simulink model "student_model_animation_2024a"  (R2024a)
settings: Solver=VariableStepAuto  StartTime=0.0  StopTime=t_sim  RelTol=1e-3
values from neighbouring files (symbols this model uses):
  L = 1    [student_lab3_model_ref.m]
undefined symbols (not defined in the file or in its folder): X, Y, Z
libraries: sm_lib x13, nesl_utility x3
settings Model: Creator=trome3  LastModifiedBy=trome3
settings ConfigComp: CovBoundaryAbsTol=1.0e-5

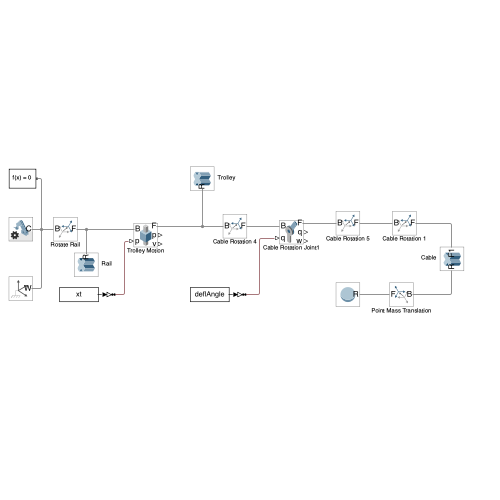
[thumbnail: Simulink's stored preview of the top-level diagram]
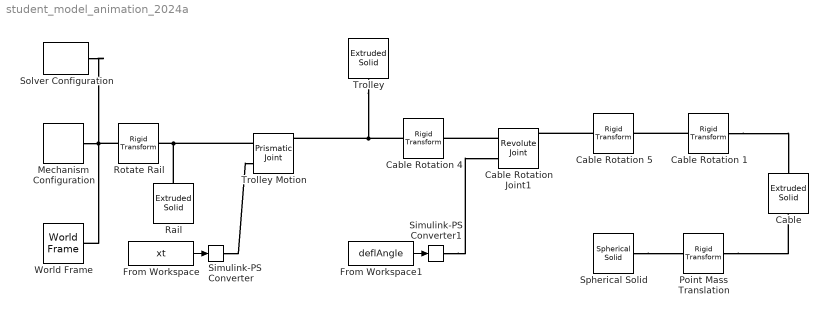
== system student_model_animation_2024a ==
  Cable : sm_lib/Body Elements/Extruded Solid  ExtrusionType=General  PolygonNumSides=1  PolygonOuterRadius=1  PolygonOuterRadiusUnits=m  ExportEntireGeometry=off  ExtrusionCrossSection=[1 1; -1 1; -1 -1; 1 -1]  ExtrusionCrossSectionUnits=cm  ExportConvexHullGeometry=off  ExtrusionLength=L  ExtrusionLengthUnits=m  InertiaType=Custom  BasedOnType=Density  Density=1000  DensityUnits=kg/m^3  Mass=0  MassUnits=kg  CenterOfMass=[0 0 0]  CenterOfMassUnits=m  MomentsOfInertia=[0 0 0]  MomentsOfInertiaUnits=kg*m^2  ProductsOfInertia=[0 0 0]  ProductsOfInertiaUnits=kg*m^2  GraphicType=FromGeometry  MarkerShape=Sphere  MarkerSize=10  GraphicVisPropType=SimpleVisualProperties  GraphicDiffuseColor=[0.5 0.5 0.5]  GraphicOpacity=1  GraphicSpecularColor=[0.5 0.5 0.5 1.0]  GraphicAmbientColor=[0.15 0.15 0.15 1.0]  GraphicEmissiveColor=[0.0 0.0 0.0 1.0]  GraphicShininess=75  DoExposeReferenceFrame=on  SerializedFrames=|
      | <Frames>
      | 
      |   <Frame>
      |     <Id>Frame1</Id>
      |     <Value>
      |       <Name>F1</Name>
      |       <Origin>
      |         <Source>GeometricFeature</Source>
      |         <FeatureName>top surface</FeatureName>
      |       </Origin>
      |       <PrimaryAxis>
      |         <DefinedDirection>+Z</DefinedDirection>
      |         <Source>ReferenceFrame</Source>
      |         <SourceDirection>+Z</SourceDirection>
      |         <FeatureName></FeatureName>
      |       </PrimaryAxis>
      |       <SecondaryAxis>
      |         <DefinedDirection>+X</DefinedDirection>
      |         <Source>ReferenceFrame</Source>
      |         <SourceDirection>+X</SourceDirection>
      |         <FeatureName></FeatureName>
      |       </SecondaryAxis>
      |     </Value>
      |   </Frame>
      | 
      | </Frames>
  Cable Rotation 1 : sm_lib/Frames and Transforms/Rigid Transform  RotationMethod=RotationSequence  FollAlignAxisA=+X  BaseAlignAxisA=+Y  FollAlignAxisB=+Y  BaseAlignAxisB=+Z  RotationStandardAxis=+Z  RotationAngle=0  RotationAngleUnits=deg  RotationArbitraryAxis=[0 0 1]  RotationSequenceAxes=FollowerAxes  RotationSequence=ZYX  RotationSequenceAngles=[0 0 -90]  RotationSequenceAnglesUnits=deg  RotationMatrix=[1 0 0;0 1 0;0 0 1]  Quaternion=[1 0 0 0]  TranslationMethod=None  TranslationCartesianOffset=[0 0 0]  TranslationCartesianOffsetUnits=m  TranslationStandardAxis=+Z  TranslationStandardOffset=L/2  TranslationStandardOffsetUnits=m  TranslationROffset=0  TranslationROffsetUnits=m  TranslationThetaOffset=0  TranslationThetaOffsetUnits=deg  TranslationZOffset=0  TranslationZOffsetUnits=m
  Cable Rotation 4 : sm_lib/Frames and Transforms/Rigid Transform  RotationMethod=RotationSequence  FollAlignAxisA=+X  BaseAlignAxisA=+Y  FollAlignAxisB=+Y  BaseAlignAxisB=+Z  RotationStandardAxis=+X  RotationAngle=0  RotationAngleUnits=deg  RotationArbitraryAxis=[0 0 1]  RotationSequenceAxes=FollowerAxes  RotationSequence=XYZ  RotationSequenceAngles=[0 90 0]  RotationSequenceAnglesUnits=deg  RotationMatrix=[1 0 0;0 1 0;0 0 1]  Quaternion=[1 0 0 0]  TranslationMethod=None  TranslationCartesianOffset=[0 0 0]  TranslationCartesianOffsetUnits=m  TranslationStandardAxis=+Z  TranslationStandardOffset=L/2  TranslationStandardOffsetUnits=m  TranslationROffset=0  TranslationROffsetUnits=m  TranslationThetaOffset=0  TranslationThetaOffsetUnits=deg  TranslationZOffset=0  TranslationZOffsetUnits=m
  Cable Rotation 5 : sm_lib/Frames and Transforms/Rigid Transform  RotationMethod=RotationSequence  FollAlignAxisA=+X  BaseAlignAxisA=+Y  FollAlignAxisB=+Y  BaseAlignAxisB=+Z  RotationStandardAxis=+X  RotationAngle=0  RotationAngleUnits=deg  RotationArbitraryAxis=[0 0 1]  RotationSequenceAxes=FollowerAxes  RotationSequence=ZYX  RotationSequenceAngles=[0 -90 0]  RotationSequenceAnglesUnits=deg  RotationMatrix=[1 0 0;0 1 0;0 0 1]  Quaternion=[1 0 0 0]  TranslationMethod=None  TranslationCartesianOffset=[0 0 0]  TranslationCartesianOffsetUnits=m  TranslationStandardAxis=+Z  TranslationStandardOffset=L/2  TranslationStandardOffsetUnits=m  TranslationROffset=0  TranslationROffsetUnits=m  TranslationThetaOffset=0  TranslationThetaOffsetUnits=deg  TranslationZOffset=0  TranslationZOffsetUnits=m
  Cable Rotation Joint1 : sm_lib/Joints/Revolute Joint  JointMode=Normal  CompositeWrenchDir=FollowerOnBase  CompositeWrenchFrame=BaseFrame  SenseConstraintForce=off  SenseConstraintTorque=off  SenseTotalForce=off  SenseTotalTorque=off  PositionTargetSpecify=off  PositionTargetPriority=High  PositionTargetValue=20  PositionTargetValueUnits=deg  VelocityTargetSpecify=off  VelocityTargetPriority=High  VelocityTargetValue=0  VelocityTargetValueUnits=deg/s  EquilibriumPosition=0  EquilibriumPositionUnits=deg  SpringStiffness=0  SpringStiffnessUnits=N*m/deg  DampingCoefficient=0  DampingCoefficientUnits=N*m/(deg/s)  LowerLimitSpecify=off  LowerLimitBound=-90  LowerLimitBoundUnits=deg  LowerLimitStiffness=1e4  LowerLimitStiffnessUnits=N*m/deg  LowerLimitDamping=10  LowerLimitDampingUnits=N*m/(deg/s)  LowerLimitTransitionRegionWidth=0.1  LowerLimitTransitionRegionWidthUnits=deg  UpperLimitSpecify=off  UpperLimitBound=90  UpperLimitBoundUnits=deg  UpperLimitStiffness=1e4  UpperLimitStiffnessUnits=N*m/deg  UpperLimitDamping=10  UpperLimitDampingUnits=N*m/(deg/s)  UpperLimitTransitionRegionWidth=0.1  UpperLimitTransitionRegionWidthUnits=deg  TorqueActuationMode=ComputedTorque  MotionActuationMode=InputMotion  SensePosition=on  SenseVelocity=on  SenseAcceleration=off  SenseTorqueForce=off  SenseLowerLimitTorqueForce=off  SenseUpperLimitTorqueForce=off
  From Workspace : FromWorkspace  VariableName=xt
  From Workspace1 : FromWorkspace  VariableName=deflAngle
  Mechanism Configuration : sm_lib/Utilities/Mechanism Configuration  UniformGravity=Constant  GravityVector=[0 0 -9.80665]  GravityVectorUnits=m/s^2  LinearizationDelta=0.001  JointModeTransitionNonlinearIterations=2
  Point Mass Translation : sm_lib/Frames and Transforms/Rigid Transform  RotationMethod=None  FollAlignAxisA=+X  BaseAlignAxisA=+Y  FollAlignAxisB=+Y  BaseAlignAxisB=+Z  RotationStandardAxis=+X  RotationAngle=0  RotationAngleUnits=deg  RotationArbitraryAxis=[0 0 1]  RotationSequenceAxes=FollowerAxes  RotationSequence=ZYX  RotationSequenceAngles=[0 -90 -90]  RotationSequenceAnglesUnits=deg  RotationMatrix=[1 0 0;0 1 0;0 0 1]  Quaternion=[1 0 0 0]  TranslationMethod=StandardAxis  TranslationCartesianOffset=[0 0 0]  TranslationCartesianOffsetUnits=m  TranslationStandardAxis=+Z  TranslationStandardOffset=-L/2  TranslationStandardOffsetUnits=m  TranslationROffset=0  TranslationROffsetUnits=m  TranslationThetaOffset=0  TranslationThetaOffsetUnits=deg  TranslationZOffset=0  TranslationZOffsetUnits=m
  Rail : sm_lib/Body Elements/Extruded Solid  ExtrusionType=General  PolygonNumSides=1  PolygonOuterRadius=1  PolygonOuterRadiusUnits=m  ExportEntireGeometry=off  ExtrusionCrossSection=[1 1; -1 1; -1 -1; 1 -1]  ExtrusionCrossSectionUnits=cm  ExportConvexHullGeometry=off  ExtrusionLength=3  ExtrusionLengthUnits=m  InertiaType=CalculateFromGeometry  BasedOnType=Density  Density=1000  DensityUnits=kg/m^3  Mass=1  MassUnits=kg  CenterOfMass=[0 0 0]  CenterOfMassUnits=m  MomentsOfInertia=[1 1 1]  MomentsOfInertiaUnits=kg*m^2  ProductsOfInertia=[0 0 0]  ProductsOfInertiaUnits=kg*m^2  GraphicType=FromGeometry  MarkerShape=Sphere  MarkerSize=10  GraphicVisPropType=SimpleVisualProperties  GraphicDiffuseColor=[0.5 0.5 0.5]  GraphicOpacity=1  GraphicSpecularColor=[0.5 0.5 0.5 1.0]  GraphicAmbientColor=[0.15 0.15 0.15 1.0]  GraphicEmissiveColor=[0.0 0.0 0.0 1.0]  GraphicShininess=75  DoExposeReferenceFrame=on  SerializedFrames=<Frames/>
  Rotate Rail : sm_lib/Frames and Transforms/Rigid Transform  RotationMethod=RotationSequence  FollAlignAxisA=+X  BaseAlignAxisA=+Y  FollAlignAxisB=+Y  BaseAlignAxisB=+Z  RotationStandardAxis=+Z  RotationAngle=0  RotationAngleUnits=deg  RotationArbitraryAxis=[0 0 1]  RotationSequenceAxes=FollowerAxes  RotationSequence=XYZ  RotationSequenceAngles=[90 0 0]  RotationSequenceAnglesUnits=deg  RotationMatrix=[1 0 0;0 1 0;0 0 1]  Quaternion=[1 0 0 0]  TranslationMethod=None  TranslationCartesianOffset=[0 0 0]  TranslationCartesianOffsetUnits=m  TranslationStandardAxis=+Z  TranslationStandardOffset=0  TranslationStandardOffsetUnits=m  TranslationROffset=0  TranslationROffsetUnits=m  TranslationThetaOffset=0  TranslationThetaOffsetUnits=deg  TranslationZOffset=0  TranslationZOffsetUnits=m
  Simulink-PS Converter : nesl_utility/Simulink-PS Converter  PhysicalDomain=network_engine_domain  SubClassName=ps_input  LeftPortType=input  RightPortType=output  PseudoPeriodic=off  Frequencies=[]  NoiseDistribution=none  NoiseParameters=[]  Unit=1  AffineConversion=off  FilteringAndDerivatives=filter  SimscapeFilterOrder=2  InputFilterTimeConstant=0.001  UdotUserProvided=0
  Simulink-PS Converter1 : nesl_utility/Simulink-PS Converter  PhysicalDomain=network_engine_domain  SubClassName=ps_input  LeftPortType=input  RightPortType=output  PseudoPeriodic=off  Frequencies=[]  NoiseDistribution=none  NoiseParameters=[]  Unit=1  AffineConversion=off  FilteringAndDerivatives=filter  SimscapeFilterOrder=2  InputFilterTimeConstant=0.001  UdotUserProvided=0
  Solver Configuration : nesl_utility/Solver Configuration  PhysicalDomain=network_engine_domain  SubClassName=solver  LeftPortType=input  RightPortType=generic  Tones=[]  Harmonics=[]  SimulateNoise=off  Profile=off  UseLocalSampling=off  EnableSwitchedLinearOptims=on  FrequencyDomain=off  UseCCode=off  RelTol=0.001  AbsTol=0.001  MinStep=1e-09  ToWorkspace=off  RevertToSquareIcSolve=off  NumHomotopyIterations=100  PhasorMode=off  PhasorModeNumHarmonics=1  ConsistencySolver=NEWTON_XTOL_AFTER_FTOL  IndexReductionMethod=DerivativeReplacement  DoDC=off  ResidualTolerance=1e-09  ConsistencyTolSource=GLOBAL  ConsistencyAbsTol=0.001  ConsistencyRelTol=0.001  ConsistencyTolFactor=0.001  UseLocalSolver=off  LocalSolverChoice=NE_BACKWARD_EULER_ADVANCER  ResolveIndetEquations=on  FunctionEvalNumThread=1  LocalSolverSampleTime=0.001  DoFixedCost=off  MaxNonlinIter=3  MaxModeIter=2  ComputeImpulses=off  ImpulseIterations=2  LinearAlgebra=auto  LinearAlgebraNumThread=0  EquationFormulation=NE_TIME_EF  DelaysMemoryBudget=1024  AutomaticFiltering=on  FilteringTimeConstant=0.001  PartitionStorageMethod=AS_NEEDED  PartitionMemoryBudget=1024  PartitionMethod=ROBUST  MultibodyUseLocalSolver=off  MultibodyLocalSolverChoice=ODE1  MultibodyLocalSolverSampleTime=0.001
  Spherical Solid : sm_lib/Body Elements/Spherical Solid  SphereRadius=0.1  SphereRadiusUnits=m  ExportEntireGeometry=off  InertiaType=PointMass  BasedOnType=Density  Density=1000  DensityUnits=kg/m^3  Mass=0  MassUnits=kg  CenterOfMass=[0 0 0]  CenterOfMassUnits=m  MomentsOfInertia=[1 1 1]  MomentsOfInertiaUnits=kg*m^2  ProductsOfInertia=[0 0 0]  ProductsOfInertiaUnits=kg*m^2  GraphicType=FromGeometry  MarkerShape=Sphere  MarkerSize=10  GraphicVisPropType=SimpleVisualProperties  GraphicDiffuseColor=[0.5 0.5 0.5]  GraphicOpacity=1  GraphicSpecularColor=[0.5 0.5 0.5 1.0]  GraphicAmbientColor=[0.15 0.15 0.15 1.0]  GraphicEmissiveColor=[0.0 0.0 0.0 1.0]  GraphicShininess=75  DoExposeReferenceFrame=on  SerializedFrames=<Frames/>
  Trolley : sm_lib/Body Elements/Extruded Solid  ExtrusionType=General  PolygonNumSides=1  PolygonOuterRadius=1  PolygonOuterRadiusUnits=m  ExportEntireGeometry=off  ExtrusionCrossSection=[0.1 0.1; -0.1 0.1; -0.1 -0.1; 0.1 -0.1]  ExtrusionCrossSectionUnits=m  ExportConvexHullGeometry=off  ExtrusionLength=0.2  ExtrusionLengthUnits=m  InertiaType=CalculateFromGeometry  BasedOnType=Density  Density=1000  DensityUnits=kg/m^3  Mass=1  MassUnits=kg  CenterOfMass=[0 0 0]  CenterOfMassUnits=m  MomentsOfInertia=[1 1 1]  MomentsOfInertiaUnits=kg*m^2  ProductsOfInertia=[0 0 0]  ProductsOfInertiaUnits=kg*m^2  GraphicType=FromGeometry  MarkerShape=Sphere  MarkerSize=10  GraphicVisPropType=SimpleVisualProperties  GraphicDiffuseColor=[0.5 0.5 0.5]  GraphicOpacity=1  GraphicSpecularColor=[0.5 0.5 0.5 1.0]  GraphicAmbientColor=[0.15 0.15 0.15 1.0]  GraphicEmissiveColor=[0.0 0.0 0.0 1.0]  GraphicShininess=75  DoExposeReferenceFrame=on  SerializedFrames=<Frames/>
  Trolley Motion : sm_lib/Joints/Prismatic Joint  JointMode=Normal  CompositeWrenchDir=FollowerOnBase  CompositeWrenchFrame=BaseFrame  SenseConstraintForce=off  SenseConstraintTorque=off  SenseTotalForce=off  SenseTotalTorque=off  PositionTargetSpecify=off  PositionTargetPriority=High  PositionTargetValue=1.5  PositionTargetValueUnits=m  VelocityTargetSpecify=off  VelocityTargetPriority=High  VelocityTargetValue=0  VelocityTargetValueUnits=m/s  EquilibriumPosition=0  EquilibriumPositionUnits=m  SpringStiffness=0  SpringStiffnessUnits=N/m  DampingCoefficient=0  DampingCoefficientUnits=N/(m/s)  LowerLimitSpecify=on  LowerLimitBound=-1.5+0.1  LowerLimitBoundUnits=m  LowerLimitStiffness=1e6  LowerLimitStiffnessUnits=N/m  LowerLimitDamping=1e3  LowerLimitDampingUnits=N/(m/s)  LowerLimitTransitionRegionWidth=1e-4  LowerLimitTransitionRegionWidthUnits=m  UpperLimitSpecify=on  UpperLimitBound=1.5-0.1  UpperLimitBoundUnits=m  UpperLimitStiffness=1e6  UpperLimitStiffnessUnits=N/m  UpperLimitDamping=1e3  UpperLimitDampingUnits=N/(m/s)  UpperLimitTransitionRegionWidth=1e-4  UpperLimitTransitionRegionWidthUnits=m  TorqueActuationMode=ComputedTorque  MotionActuationMode=InputMotion  SensePosition=on  SenseVelocity=on  SenseAcceleration=off  SenseTorqueForce=off  SenseLowerLimitTorqueForce=off  SenseUpperLimitTorqueForce=off
  World Frame : sm_lib/Frames and Transforms/World Frame
  wires:
  From Workspace1/1 -> Simulink-PS Converter1/1
  From Workspace/1 -> Simulink-PS Converter/1
  connections:
  Mechanism Configuration/RConn1 -- Rotate Rail/LConn1 -- Solver Configuration/RConn1 -- World Frame/RConn1
  Rail/RConn1 -- Trolley Motion/LConn1 -- Rotate Rail/RConn1
  Trolley/RConn1 -- Trolley Motion/RConn1 -- Cable Rotation 4/LConn1
  Point Mass Translation/LConn1 -- Cable/RConn1
  Spherical Solid/RConn1 -- Point Mass Translation/RConn1
  Cable Rotation Joint1/LConn1 -- Cable Rotation 4/RConn1
  Cable Rotation 5/LConn1 -- Cable Rotation Joint1/RConn1
  Cable Rotation 1/LConn1 -- Cable Rotation 5/RConn1
  Cable Rotation 1/RConn1 -- Cable/LConn1
  Simulink-PS Converter/RConn1 -- Trolley Motion/LConn2
  Simulink-PS Converter1/RConn1 -- Cable Rotation Joint1/LConn2
